simulink model "mod_pm"  (R2024b)
settings: Solver=FixedStepDiscrete  StartTime=0.0  StopTime=0.05  FixedStep=5e-06  RelTol=1e-3
model workspace (MAT data in the model file):
  bp = 1.5
  fc = 10000
  fm = 1000
  fs = 200000
  hpost = [-1.25061059478e-19 -3.24125186585e-05 -6.55214055151e-05 -9.93614444025e-05 -0.000133925361151 -0.000169142005337 -0.000204855936976 -0.00024080932373 -0.0002766270145 -0.000311805588382 -0.000345707084751 -0.000377558002721 ... (201 elements, 1x201)]
  hpre = [-2.4993987069e-19 -6.42670110592e-05 -0.000126833377255 -0.000184633240487 -0.000234548351952 -0.000273478101959 -0.00029844948245 -0.000306771591638 -0.000296232329902 -0.000265327256793 -0.000213503048842 -0.000141391531522 ... (201 elements, 1x201)]
  phi = 0.7
  sigma2 = 0.02
settings Model: Creator=runner  LastModifiedBy=runner

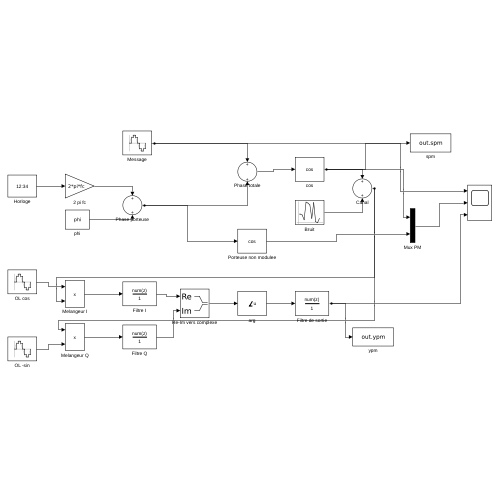
[thumbnail: Simulink's stored preview of the top-level diagram]
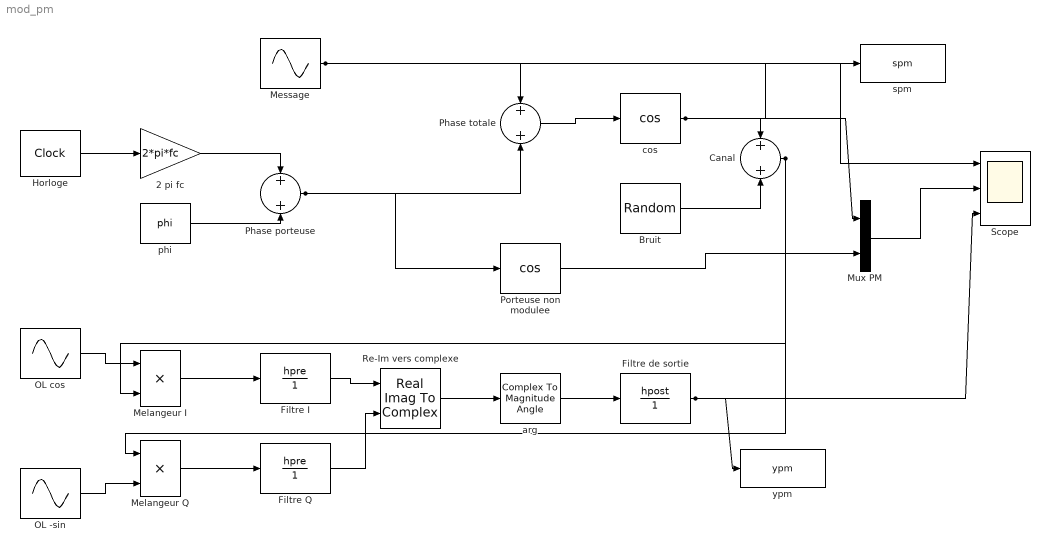
== system mod_pm ==
  2 pi fc : Gain  Gain=2*pi*fc
  Bruit : RandomNumber  Variance=sigma2  Seed=1  SampleTime=1/fs
  Canal : Sum
  Filtre I : DiscreteFilter  Numerator=hpre  Denominator=1
  Filtre Q : DiscreteFilter  Numerator=hpre  Denominator=1
  Filtre de sortie : DiscreteFilter  Numerator=hpost  Denominator=1
  Horloge : DigitalClock  SampleTime=1/fs
  Melangeur I : Product
  Melangeur Q : Product
  Message : Sin  Amplitude=bp  Frequency=2*pi*fm  Phase=pi/2  SampleTime=1/fs
  Mux PM : Mux  Inputs=2
  OL -sin : Sin  Amplitude=-2  Frequency=2*pi*fc  SampleTime=1/fs
  OL cos : Sin  Amplitude=2  Frequency=2*pi*fc  Phase=pi/2  SampleTime=1/fs
  Phase porteuse : Sum
  Phase totale : Sum
  Porteuse non modulee : Trigonometry  Operator=cos
  Re-Im vers complexe : RealImagToComplex
  Scope : Scope  NumInputPorts=3
  arg : ComplexToMagnitudeAngle  Output=Angle
  cos : Trigonometry  Operator=cos
  phi : Constant  Value=phi
  spm : ToWorkspace  VariableName=spm  SampleTime=-1
  ypm : ToWorkspace  VariableName=ypm  SampleTime=-1
  wires:
  Horloge/1 -> 2 pi fc/1
  2 pi fc/1 -> Phase porteuse/1
  phi/1 -> Phase porteuse/2
  Message/1 -> Phase totale/1, Scope/1
  Phase porteuse/1 -> Phase totale/2, Porteuse non modulee/1
  Phase totale/1 -> cos/1
  cos/1 -> Canal/1, Mux PM/1, spm/1
  Bruit/1 -> Canal/2
  Porteuse non modulee/1 -> Mux PM/2
  OL cos/1 -> Melangeur I/1
  Canal/1 -> Melangeur I/2, Melangeur Q/1
  OL -sin/1 -> Melangeur Q/2
  Melangeur I/1 -> Filtre I/1
  Melangeur Q/1 -> Filtre Q/1
  Filtre I/1 -> Re-Im vers complexe/1
  Filtre Q/1 -> Re-Im vers complexe/2
  Re-Im vers complexe/1 -> arg/1
  arg/1 -> Filtre de sortie/1
  Filtre de sortie/1 -> ypm/1, Scope/3
  Mux PM/1 -> Scope/2
